simulink model "trucksim_different_condition"  (R2023b)
settings: Solver=FixedStepAuto  StartTime=0.0  StopTime=25  FixedStep=0.001  RelTol=1e-3  EnableMultiTasking=on
values from neighbouring files (symbols this model uses):
  g = 9.8    [Truck_simulate_different_condition.m]
  m = m_sprung + m_load + m_unsprung    (= 10505)    [Truck_simulate_different_condition.m]
  r = 0.510    (= 0.51)    [Truck_simulate_different_condition.m]
  vx0 = 5    [Truck_simulate_different_condition.m]
  vy0 = 0    [Truck_simulate_different_condition.m]
  w0 = vx0 / r    (= 9.80392156863)    [Truck_simulate_different_condition.m]
  wz0 = 0    [Truck_simulate_different_condition.m]
undefined symbols (not defined in the file or in its folder): A, Bf, Br, Cd, Cs_f, f, He, hg, Hp, I_tire, Ix, Iy, Iz, ks_f, kw, L, Lf, Lr, mb, mw, p
libraries: SignalEditorBlockLib x6, Solver_SF x1
(part 1 of 4)
settings Model: Creator=dzY  LastModifiedBy=Admin
settings DataIOCC: SaveFormat=Array  ReturnWorkspaceOutputs=off
settings OptimizationCC: LifeSpan=inf
settings DebuggingCC: SolverPrmCheckMsg=warning  UnconnectedInputMsg=warning  UnconnectedOutputMsg=warning  UnconnectedLineMsg=warning  SFUnexpectedBacktrackingDiag=warning  SFNoUnconditionalDefaultTransitionDiag=warning  SFExecutionAtInitializationDiag=none  ArithmeticOperatorsInVariantConditions=warning
settings HardwareCC: ProdBitPerPointer=32  ProdBitPerSizeT=32  ProdBitPerPtrDiffT=32  ProdLargestAtomicFloat=None  ProdIntDivRoundTo=Undefined  ProdEndianess=Unspecified  ProdWordSize=32  ProdHWDeviceType=32-bit Generic
settings ModelReferenceCC: EnableRefExpFcnMdlSchedulingChecks=on  PropagateSignalLabelsOutOfModel=off
settings SFSimCC: SimUseLocalCustomCode=off  CustomCodeUndefinedFunction=UseInterfaceOnly
settings RTWCC: RTWUseLocalCustomCode=off
settings CodeAppCC: StateflowObjectComments=on
settings GRTTargetCC: TargetLangStandard=C89/C90 (ANSI)
settings ConfigComp: CovMetricSettings=dw  CovSaveCumulativeToWorkspaceVar=on  CovSaveSingleToWorkspaceVar=on  CovExternalEMLEnable=off  CovSFcnEnable=off

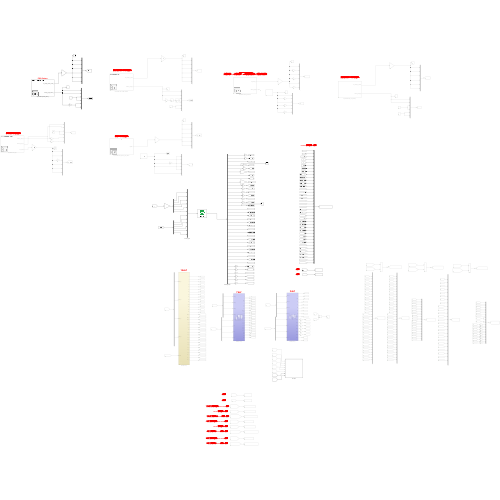
[thumbnail: Simulink's stored preview of the top-level diagram]
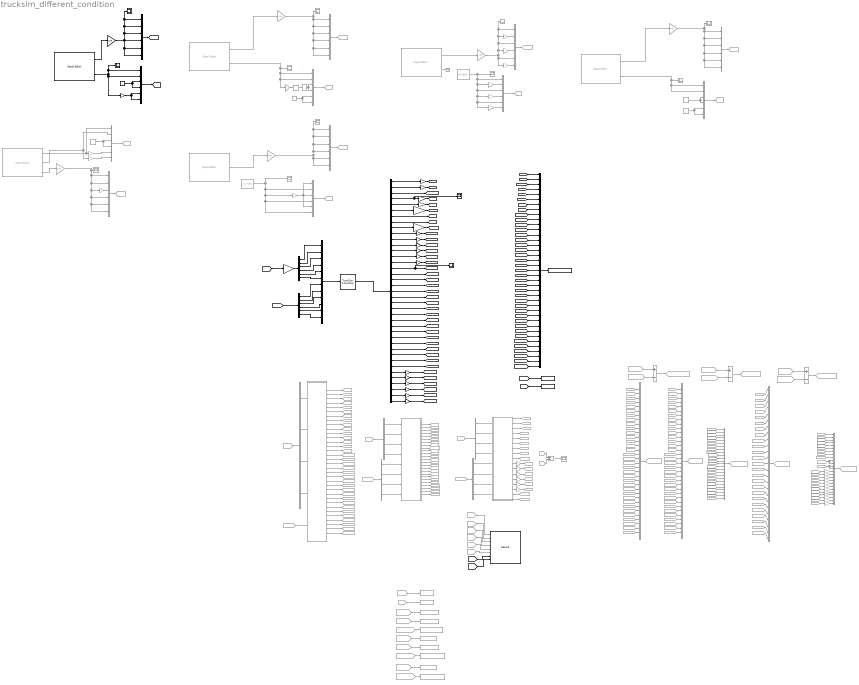
== system trucksim_different_condition ==
  note: FRO Pattern
  note: 原地掉头控制输入
  note: 7dof
  note: 4维度
  note: 4维度
  note: 十四自由度模型输出18+4+12=34维度
  note: carsim模型输出34维度
  note: 十四自由度模型与carsim残差34维度
  note: carsim模型输出25维度
  note: 七自由度模型与carsim残差25维度
  note: 七自由度模型输出18+4+12=25维度
  note: 14dof
  note: 3dof
  note: 三自由度模型与carsim残差25维度
  note: 三自由度模型输出18+4+12=25维度
  note: 6维度
  note: trucksim模型输出39维度
  note: 6维度
  note: 前中轴转向工况控制输入
  note: 蟹形工况控制输入
  note: 横移工况控制输入
      | (左侧左转90，右侧右转90，左侧前进转矩，右侧后退转矩)
  note: 仅前轴转向工况控制输入
  14DOF整车模型 : Subsystem  Commented=on
  3DOF整车模型 : Subsystem  Commented=on
  7DOF整车模型 : Subsystem  Commented=on
  Add{,1..3} (4 alike) : Sum  Commented=on  Inputs=+-
  Constant{,3,5..6} (4 alike) : Constant  Commented=on  Value=0
  Constant1 : Constant  Value=0
  Constant2 : Constant  Commented=on  Value=3.1415/2
  Constant4 : Constant  Commented=on  Value=3.14159/2
  Demux{,2,4..6} (5 alike) : Demux  Commented=on
  Demux1 : Demux  Outputs=6
  Demux3 : Demux  Outputs=6
  From{,32,82,89} (4 alike) : From  Commented=on  GotoTag=delta_act
  From1 : From  Commented=on  GotoTag=x_14dof
  From10 : From  Commented=on  GotoTag=ay_14dof
  From100 : From  Commented=on  GotoTag=Fy_fl_7dof
  From101 : From  Commented=on  GotoTag=Fz_fl_7dof
  From102 : From  Commented=on  GotoTag=Fx_fr_7dof
  From103 : From  Commented=on  GotoTag=Fy_fr_7dof
  From104 : From  Commented=on  GotoTag=Fz_fr_7dof
  From105 : From  Commented=on  GotoTag=Fx_rl_7dof
  From106 : From  Commented=on  GotoTag=Fy_rl_7dof
  From107 : From  Commented=on  GotoTag=Fz_rl_7dof
  From108 : From  Commented=on  GotoTag=Fx_rr_7dof
  From109 : From  Commented=on  GotoTag=Fy_rr_7dof
  From11 : From  Commented=on  GotoTag=az_14dof
  From110 : From  Commented=on  GotoTag=Fz_rr_7dof
  From111 : From  Commented=on  GotoTag=Fx_fl_carsim
  From112 : From  Commented=on  GotoTag=Fy_fl_carsim
  From113 : From  Commented=on  GotoTag=x_carsim
  From114 : From  Commented=on  GotoTag=y_carsim
  From115 : From  Commented=on  GotoTag=state_7dof_25d
  From116 : From  Commented=on  GotoTag=vx_carsim
  From117 : From  Commented=on  GotoTag=state_carsim_25d
  From118 : From  Commented=on  GotoTag=vy_carsim
  From119 : From  Commented=on  GotoTag=ax_carsim
  From12 : From  Commented=on  GotoTag=roll_14dof
  From120 : From  Commented=on  GotoTag=ay_carsim
  From121 : From  Commented=on  GotoTag=state_7dof_25d
  From122 : From  Commented=on  GotoTag=state_residual_7dof_25d
  From123 : From  Commented=on  GotoTag=state_carsim_25d
  From124 : From  Commented=on  GotoTag=yaw_carsim
  From125 : From  Commented=on  GotoTag=Fy_f_3dof
  From126 : From  Commented=on  GotoTag=Fz_f_3dof
  From127 : From  Commented=on  GotoTag=wz_carsim
  From128 : From  Commented=on  GotoTag=Fy_r_3dof
  From129 : From  Commented=on  GotoTag=Fz_r_3dof
  From13 : From  Commented=on  GotoTag=phi_14dof
  From130 : From  Commented=on  GotoTag=beta_z_carsim
  From131 : From  Commented=on  GotoTag=w_fl_carsim
  From132 : From  Commented=on  GotoTag=w_fr_carsim
  From133 : From  Commented=on  GotoTag=w_rl_carsim
  From134 : From  Commented=on  GotoTag=w_rr_carsim
  From135 : From  Commented=on  GotoTag=Fz_fl_carsim
  From136 : From  Commented=on  GotoTag=Fx_fr_carsim
  From137 : From  Commented=on  GotoTag=Fy_fr_carsim
  From138 : From  Commented=on  GotoTag=Fz_fr_carsim
  From139 : From  Commented=on  GotoTag=Fx_rl_carsim
  From140 : From  Commented=on  GotoTag=Fy_rl_carsim
  From141 : From  Commented=on  GotoTag=Fz_rl_carsim
  From142 : From  Commented=on  GotoTag=Fx_rr_carsim
  From143 : From  Commented=on  GotoTag=Fy_rr_carsim
  From144 : From  Commented=on  GotoTag=Fz_rr_carsim
  From145 : From  Commented=on  GotoTag=Fx_r_3dof
  From146 : From  Commented=on  GotoTag=Fy_r_3dof
  From147 : From  Commented=on  GotoTag=Fz_r_3dof
  From148 : From  Commented=on  GotoTag=Fx_r_3dof
  From149 : From  Commented=on  GotoTag=w_f_3dof
  From15 : From  Commented=on  GotoTag=yaw_14dof
  From150 : From  Commented=on  GotoTag=state_3dof_25d
  From151 : From  Commented=on  GotoTag=w_r_3dof
  From152 : From  Commented=on  GotoTag=state_3dof_25d
  From153 : From  Commented=on  GotoTag=x_3dof
  From154 : From  Commented=on  GotoTag=y_3dof
  From155 : From  Commented=on  GotoTag=yaw_3dof
  From156 : From  Commented=on  GotoTag=vx_3dof
  From157 : From  Commented=on  GotoTag=vy_3dof
  From158 : From  Commented=on  GotoTag=wz_3dof
  From159 : From  Commented=on  GotoTag=ax_3dof
  From16 : From  Commented=on  GotoTag=wx_14dof
  From160 : From  Commented=on  GotoTag=ay_3dof
  From161 : From  Commented=on  GotoTag=beta_z_3dof
  From162 : From  Commented=on  GotoTag=Fx_f_3dof
  From163 : From  Commented=on  GotoTag=state_carsim_25d
  From164 : From  Commented=on  GotoTag=state_residual_3dof_25d
  From165 : From  Commented=on  GotoTag=x_14dof
  From166 : From  Commented=on  GotoTag=y_14dof
  From167 : From  Commented=on  GotoTag=x_7dof
  From168 : From  Commented=on  GotoTag=y_7dof
  From169 : From  Commented=on  GotoTag=x_3dof
  From17 : From  Commented=on  GotoTag=wy_14dof
  From170 : From  Commented=on  GotoTag=y_3dof
  From173 : From  Commented=on  GotoTag=vx_14dof
  From174 : From  Commented=on  GotoTag=vx_carsim
  From18 : From  Commented=on  GotoTag=wz_14dof
  From19 : From  Commented=on  GotoTag=beta_x_14dof
  From2 : From  Commented=on  GotoTag=y_14dof
  From20 : From  Commented=on  GotoTag=beta_y_14dof
  From21 : From  Commented=on  GotoTag=beta_z_14dof
  From22 : From  Commented=on  GotoTag=w_fl_14dof
  From23 : From  Commented=on  GotoTag=w_fr_14dof
  From24 : From  Commented=on  GotoTag=w_rl_14dof
  From25 : From  Commented=on  GotoTag=w_rr_14dof
  From26 : From  Commented=on  GotoTag=state_carsim_34d
  From27 : From  Commented=on  GotoTag=state_14dof_34d
  From28 : From  Commented=on  GotoTag=w_fl_7dof
  From29 : From  Commented=on  GotoTag=w_fr_7dof
  From30 : From  Commented=on  GotoTag=w_rl_7dof
  From{4,31,81,88} (4 alike) : From  Commented=on  GotoTag=T_motor
  From33 : From  Commented=on  GotoTag=Fy_f_3dof
  From34 : From  Commented=on  GotoTag=Fz_f_3dof
  From35 : From  Commented=on  GotoTag=Fx_fl_carsim
  From36 : From  Commented=on  GotoTag=Fy_fl_carsim
  From37 : From  Commented=on  GotoTag=x_carsim
  From38 : From  Commented=on  GotoTag=y_carsim
  From39 : From  Commented=on  GotoTag=z_carsim
  From40 : From  Commented=on  GotoTag=vx_carsim
  From41 : From  Commented=on  GotoTag=vz_carsim
  From42 : From  Commented=on  GotoTag=vy_carsim
  From43 : From  Commented=on  GotoTag=ax_carsim
  From44 : From  Commented=on  GotoTag=ay_carsim
  From45 : From  Commented=on  GotoTag=az_carsim
  From46 : From  Commented=on  GotoTag=roll_carsim
  From47 : From  Commented=on  GotoTag=phi_carsim
  From48 : From  Commented=on  GotoTag=yaw_carsim
  From49 : From  Commented=on  GotoTag=wx_carsim
  From5 : From  Commented=on  GotoTag=z_14dof
  From50 : From  Commented=on  GotoTag=wy_carsim
  From51 : From  Commented=on  GotoTag=wz_carsim
  From52 : From  Commented=on  GotoTag=beta_x_carsim
  From53 : From  Commented=on  GotoTag=beta_y_carsim
  From54 : From  Commented=on  GotoTag=beta_z_carsim
  From55 : From  Commented=on  GotoTag=w_fl_carsim
  From56 : From  Commented=on  GotoTag=w_fr_carsim
  From57 : From  Commented=on  GotoTag=w_rl_carsim
  From58 : From  Commented=on  GotoTag=w_rr_carsim
  From59 : From  Commented=on  GotoTag=Fz_fl_carsim
  From6 : From  Commented=on  GotoTag=vx_14dof
  From60 : From  Commented=on  GotoTag=Fx_fr_carsim
  From61 : From  Commented=on  GotoTag=Fy_fr_carsim
  From62 : From  Commented=on  GotoTag=Fz_fr_carsim
  From63 : From  Commented=on  GotoTag=Fx_rl_carsim
  From64 : From  Commented=on  GotoTag=Fy_rl_carsim
  From65 : From  Commented=on  GotoTag=Fz_rl_carsim
  From66 : From  Commented=on  GotoTag=Fx_rr_carsim
  From67 : From  Commented=on  GotoTag=Fy_rr_carsim
  From68 : From  Commented=on  GotoTag=Fz_rr_carsim
  From69 : From  Commented=on  GotoTag=Fx_fl_14dof
  From7 : From  Commented=on  GotoTag=vy_14dof
  From70 : From  Commented=on  GotoTag=Fy_fl_14dof
  From71 : From  Commented=on  GotoTag=Fz_fl_14dof
  From72 : From  Commented=on  GotoTag=Fx_fr_14dof
  From73 : From  Commented=on  GotoTag=Fy_fr_14dof
  From74 : From  Commented=on  GotoTag=Fz_fr_14dof
  From75 : From  Commented=on  GotoTag=Fx_rl_14dof
  From76 : From  Commented=on  GotoTag=Fy_rl_14dof
  From77 : From  Commented=on  GotoTag=Fz_rl_14dof
  From78 : From  Commented=on  GotoTag=Fx_rr_14dof
  From79 : From  Commented=on  GotoTag=Fy_rr_14dof
  From8 : From  Commented=on  GotoTag=vz_14dof
  From80 : From  Commented=on  GotoTag=Fz_rr_14dof
  From83 : From  Commented=on  GotoTag=state_14dof_34d
  From84 : From  Commented=on  GotoTag=state_residual_14dof_34d
  From85 : From  Commented=on  GotoTag=w_rr_7dof
  From86 : From  Commented=on  GotoTag=Fx_f_3dof
  From87 : From  Commented=on  GotoTag=state_carsim_34d
  From9 : From  Commented=on  GotoTag=ax_14dof
  From90 : From  Commented=on  GotoTag=x_7dof
  From91 : From  Commented=on  GotoTag=y_7dof
  From92 : From  Commented=on  GotoTag=yaw_7dof
  From93 : From  Commented=on  GotoTag=vx_7dof
  From94 : From  Commented=on  GotoTag=vy_7dof
  From95 : From  Commented=on  GotoTag=wz_7dof
  From96 : From  Commented=on  GotoTag=ax_7dof
  From97 : From  Commented=on  GotoTag=ay_7dof
  From98 : From  Commented=on  GotoTag=beta_z_7dof
  From99 : From  Commented=on  GotoTag=Fx_fl_7dof
  Gain : Gain  Gain=1/3.6
  Gain{1,39,43,46,48..53} (10 alike) : Gain  Commented=on  Gain=-1
  Gain{8..10,12,35..38} (8 alike) : Gain  Gain=3.1415/180
  Gain{11,18..22} (6 alike) : Gain  Commented=on  Gain=2
  Gain{3,6,13..16} (6 alike) : Gain  Gain=3.1415/30
  Gain17 : Gain  Gain=180/3.1415
  Gain2 : Gain  Gain=1/3.6
  Gain{23..34,45} (13 alike) : Gain  Commented=on  Gain=0.5
  Gain4 : Gain  Gain=9.8
  Gain40 : Gain  Gain=-1
  Gain{7,41,44,47,54} (5 alike) : Gain  Commented=on  Gain=100
  Gain42 : Gain  Gain=100
  Gain5 : Gain  Gain=9.8
  Goto{,127,129,131,133} (5 alike) : Goto  Commented=on  GotoTag=delta_act
  Goto1 : Goto  Commented=on  GotoTag=w_fl_14dof
  Goto100 : Goto  Commented=on  GotoTag=state_residual_7dof_25d
  Goto101 : Goto  Commented=on  GotoTag=wz_3dof
  Goto102 : Goto  Commented=on  GotoTag=ax_3dof
  Goto103 : Goto  Commented=on  GotoTag=vy_3dof
  Goto104 : Goto  Commented=on  GotoTag=vx_3dof
  Goto105 : Goto  Commented=on  GotoTag=Fx_f_3dof
  Goto106 : Goto  Commented=on  GotoTag=Fy_f_3dof
  Goto107 : Goto  Commented=on  GotoTag=Fz_f_3dof
  Goto108 : Goto  Commented=on  GotoTag=state_3dof_25d
  Goto109 : Goto  Commented=on  GotoTag=state_residual_3dof_25d
  Goto111 : Goto  Commented=on  GotoTag=Fx_r_3dof
  Goto112 : Goto  Commented=on  GotoTag=Fy_r_3dof
  Goto113 : Goto  Commented=on  GotoTag=Fz_r_3dof
  Goto117 : Goto  Commented=on  GotoTag=ay_3dof
  Goto118 : Goto  Commented=on  GotoTag=beta_z_3dof
  Goto119 : Goto  Commented=on  GotoTag=x_3dof
  Goto120 : Goto  Commented=on  GotoTag=y_3dof
  Goto121 : Goto  Commented=on  GotoTag=yaw_3dof
  Goto122 : Goto  Commented=on  GotoTag=w_f_3dof
  Goto124 : Goto  Commented=on  GotoTag=w_r_3dof
  Goto{38,128,130,132,134} (5 alike) : Goto  Commented=on  GotoTag=T_motor
  Goto2 : Goto  Commented=on  GotoTag=x_14dof
  Goto3 : Goto  Commented=on  GotoTag=y_14dof
  Goto31 : Goto  Commented=on  GotoTag=state_carsim_34d
  Goto32 : Goto  Commented=on  GotoTag=state_14dof_34d
  Goto33 : Goto  Commented=on  GotoTag=state_residual_14dof_34d
  Goto34 : Goto  Commented=on  GotoTag=wz_7dof
  Goto4 : Goto  Commented=on  GotoTag=z_14dof
  Goto48 : Goto  Commented=on  GotoTag=Fx_fl_14dof
  Goto49 : Goto  Commented=on  GotoTag=vy_14dof
  Goto5 : Goto  Commented=on  GotoTag=vx_14dof
  Goto50 : Goto  Commented=on  GotoTag=vz_14dof
  Goto51 : Goto  Commented=on  GotoTag=ax_14dof
  Goto52 : Goto  Commented=on  GotoTag=ay_14dof
  Goto53 : Goto  Commented=on  GotoTag=az_14dof
  Goto54 : Goto  Commented=on  GotoTag=roll_14dof
  Goto55 : Goto  Commented=on  GotoTag=phi_14dof
  Goto56 : Goto  Commented=on  GotoTag=yaw_14dof
  Goto57 : Goto  Commented=on  GotoTag=wx_14dof
  Goto58 : Goto  Commented=on  GotoTag=wy_14dof
  Goto59 : Goto  Commented=on  GotoTag=wz_14dof
  Goto6 : Goto  Commented=on  GotoTag=w_fr_14dof
  Goto60 : Goto  Commented=on  GotoTag=beta_x_14dof
  Goto61 : Goto  Commented=on  GotoTag=beta_y_14dof
  Goto62 : Goto  Commented=on  GotoTag=beta_z_14dof
  Goto63 : Goto  Commented=on  GotoTag=Fy_fl_14dof
  Goto64 : Goto  Commented=on  GotoTag=Fz_fl_14dof
  Goto65 : Goto  Commented=on  GotoTag=Fx_fr_14dof
  Goto66 : Goto  Commented=on  GotoTag=Fy_fr_14dof
  Goto67 : Goto  Commented=on  GotoTag=Fz_fr_14dof
  Goto68 : Goto  Commented=on  GotoTag=Fx_rl_14dof
  Goto69 : Goto  Commented=on  GotoTag=Fy_rl_14dof
  Goto7 : Goto  Commented=on  GotoTag=w_rl_14dof
  Goto70 : Goto  Commented=on  GotoTag=Fz_rl_14dof
  Goto71 : Goto  Commented=on  GotoTag=Fx_rr_14dof
  Goto72 : Goto  Commented=on  GotoTag=Fy_rr_14dof
  Goto73 : Goto  Commented=on  GotoTag=Fz_rr_14dof
  Goto74 : Goto  Commented=on  GotoTag=ax_7dof
  Goto75 : Goto  Commented=on  GotoTag=vy_7dof
  Goto76 : Goto  Commented=on  GotoTag=vx_7dof
  Goto77 : Goto  Commented=on  GotoTag=Fx_fl_7dof
  Goto78 : Goto  Commented=on  GotoTag=Fy_fl_7dof
  Goto79 : Goto  Commented=on  GotoTag=Fz_fl_7dof
  Goto8 : Goto  Commented=on  GotoTag=w_rr_14dof
  Goto80 : Goto  Commented=on  GotoTag=Fx_fr_7dof
  Goto81 : Goto  Commented=on  GotoTag=Fy_fr_7dof
  Goto82 : Goto  Commented=on  GotoTag=Fz_fr_7dof
  Goto83 : Goto  Commented=on  GotoTag=Fx_rl_7dof
  Goto84 : Goto  Commented=on  GotoTag=Fy_rl_7dof
  Goto85 : Goto  Commented=on  GotoTag=Fz_rl_7dof
  Goto86 : Goto  Commented=on  GotoTag=Fx_rr_7dof
  Goto87 : Goto  Commented=on  GotoTag=Fy_rr_7dof
  Goto88 : Goto  Commented=on  GotoTag=Fz_rr_7dof
  Goto89 : Goto  Commented=on  GotoTag=ay_7dof
  Goto90 : Goto  Commented=on  GotoTag=beta_z_7dof
  Goto91 : Goto  Commented=on  GotoTag=x_7dof
  Goto92 : Goto  Commented=on  GotoTag=y_7dof
  Goto93 : Goto  Commented=on  GotoTag=yaw_7dof
  Goto94 : Goto  Commented=on  GotoTag=state_7dof_25d
  Goto95 : Goto  Commented=on  GotoTag=w_fl_7dof
  Goto96 : Goto  Commented=on  GotoTag=w_fr_7dof
  Goto97 : Goto  Commented=on  GotoTag=w_rl_7dof
  Goto98 : Goto  Commented=on  GotoTag=w_rr_7dof
  Goto99 : Goto  Commented=on  GotoTag=state_carsim_25d
  Mux{,4,10..17} (10 alike) : Mux  Commented=on  Inputs=6
  Mux1 : Mux  Commented=on  Inputs=34
  Mux2 : Mux  Commented=on  Inputs=34
  Mux3 : Mux  Commented=on  Inputs=25
  Mux5 : Mux  Commented=on  Inputs=25
  Mux6 : Mux  Commented=on  Inputs=25
  Mux7 : Mux  Inputs=39
  Mux8 : Mux  Inputs=6
  Mux9 : Mux  Inputs=6
  Scope{,4..5,7..13} (10 alike) : Scope  Commented=on
  Scope{1..3,6} (4 alike) : Scope
  Signal Editor-front_middle_steering : SignalEditorBlockLib/Signal Editor  Commented=on  FileName=D:\YRJ_Workspace\Dynamic_Model_with_NN_truck\data\trucksim\different_scenarios\scenarios_input\Scenario-input_front_middle_steering_v1.mat  ActiveScenario=Scenario_snake_deacc_5m_s_16  ActiveSignal=tire_torque_4_deacc  IsBus=off  OutputBusObjectStr=Bus: BusObject  SampleTime=0  ZeroCross=off  OutputAfterFinalValue=Setting to zero  Unit=inherit  PreserveSignalName=on  ApplySigPropsToAllScenarios=on  ApplySigPropsToAllSignals=on
  Signal Editor-lateral_movement : SignalEditorBlockLib/Signal Editor  Commented=on  FileName=D:\YRJ_Workspace\Dynamic_Model_with_NN_truck\data\trucksim\different_scenarios\scenarios_input\Scenario-input_lateral_movement_v1.mat  ActiveScenario=Scenario_lateral_movement_6  ActiveSignal=tire_torque_6  IsBus=off  OutputBusObjectStr=Bus: BusObject  SampleTime=0  ZeroCross=off  OutputAfterFinalValue=Setting to zero  Unit=inherit  PreserveSignalName=on  ApplySigPropsToAllScenarios=on  ApplySigPropsToAllSignals=on
  Signal Editor-only_front_steering : SignalEditorBlockLib/Signal Editor  Commented=on  FileName=D:\YRJ_Workspace\Dynamic_Model_with_NN_truck\data\trucksim\different_scenarios\scenarios_input\Scenario-input_front_middle_steering_v1.mat  ActiveScenario=Scenario_snake_deacc_5m_s_16  ActiveSignal=tire_torque_4_deacc  IsBus=off  OutputBusObjectStr=Bus: BusObject  SampleTime=0  ZeroCross=off  OutputAfterFinalValue=Setting to zero  Unit=inherit  PreserveSignalName=on  ApplySigPropsToAllScenarios=on  ApplySigPropsToAllSignals=on
  Signal Editor-opposite_steering : SignalEditorBlockLib/Signal Editor  FileName=D:\YRJ_Workspace\Dynamic_Model_with_NN_truck\data\trucksim\different_scenarios\scenarios_input\Scenario-input_snake_rollover_v2_5m_s.mat  ActiveScenario=Scenario_snake_rollover_5m_s_1  ActiveSignal=tire_torque_rollover_const_1  IsBus=off  OutputBusObjectStr=Bus: BusObject  SampleTime=0  ZeroCross=off  OutputAfterFinalValue=Setting to zero  Unit=inherit  PreserveSignalName=on  ApplySigPropsToAllScenarios=on  ApplySigPropsToAllSignals=on
  Signal Editor-same_steering_crab_motion : SignalEditorBlockLib/Signal Editor  Commented=on  FileName=D:\YRJ_Workspace\Dynamic_Model_with_NN_truck\data\trucksim\different_scenarios\scenarios_input\Scenario-input_same_steering_lateral_movement_v1.mat  ActiveScenario=Scenario_lateral_movement_6  ActiveSignal=tire_torque_6  IsBus=off  OutputBusObjectStr=Bus: BusObject  SampleTime=0  ZeroCross=off  OutputAfterFinalValue=Setting to zero  Unit=inherit  PreserveSignalName=on  ApplySigPropsToAllScenarios=on  ApplySigPropsToAllSignals=on
  Signal Editor-tank_turn : SignalEditorBlockLib/Signal Editor  Commented=on  FileName=D:\YRJ_Workspace\Dynamic_Model_with_NN_truck\data\trucksim\different_scenarios\scenarios_input\Scenario-input_tank_turn_v1.mat  ActiveScenario=Scenario_tank_turn_1500Nm  ActiveSignal=steering_angle_fl  IsBus=off  OutputBusObjectStr=Bus: BusObject  SampleTime=0  ZeroCross=off  OutputAfterFinalValue=Setting to zero  Unit=inherit  PreserveSignalName=on  ApplySigPropsToAllScenarios=on  ApplySigPropsToAllSignals=on
  Terminator1 : Terminator  Commented=on
  To Workspace1 : ToWorkspace  Commented=on  VariableName=T_motor_out  SaveFormat=Timeseries  SampleTime=-1
  To Workspace10 : ToWorkspace  Commented=on  VariableName=Vehicle_state_residual_3dof_25d_out  SaveFormat=Timeseries  SampleTime=-1
  To Workspace11 : ToWorkspace  VariableName=Vehicle_state_trucksim_39d_out  SaveFormat=Timeseries  SampleTime=-1
  To Workspace12 : ToWorkspace  VariableName=T_motor_out  SaveFormat=Timeseries  SampleTime=-1
  To Workspace13 : ToWorkspace  VariableName=Delta_act_out  SaveFormat=Timeseries  SampleTime=-1
  To Workspace2 : ToWorkspace  Commented=on  VariableName=Vehicle_state_7dof_25d_out  SaveFormat=Timeseries  SampleTime=-1
  To Workspace3 : ToWorkspace  Commented=on  VariableName=Delta_act_out  SaveFormat=Timeseries  SampleTime=-1
  To Workspace4 : ToWorkspace  Commented=on  VariableName=Vehicle_state_14dof_34d_out  SaveFormat=Timeseries  SampleTime=-1
  To Workspace5 : ToWorkspace  Commented=on  VariableName=Vehicle_state_residual_14dof_34d_out  SaveFormat=Timeseries  SampleTime=-1
  To Workspace6 : ToWorkspace  Commented=on  VariableName=Vehicle_state_carsim_34d_out  SaveFormat=Timeseries  SampleTime=-1
  To Workspace7 : ToWorkspace  Commented=on  VariableName=Vehicle_state_residual_7dof_25d_out  SaveFormat=Timeseries  SampleTime=-1
  To Workspace8 : ToWorkspace  Commented=on  VariableName=Vehicle_state_carsim_25d_out  SaveFormat=Timeseries  SampleTime=-1
  To Workspace9 : ToWorkspace  Commented=on  VariableName=Vehicle_state_3dof_25d_out  SaveFormat=Timeseries  SampleTime=-1
  Trigonometric Function : Trigonometry  Commented=on  Operator=tan
  Trigonometric Function1 : Trigonometry  Commented=on  Operator=atan
  TruckSim S-Function : Solver_SF/TruckSim S-Function  Priority=1  SIMFILE=simfile.sim
      settings: SourceProductName=TruckSim S-Function
  Trucksim_Input : Mux  Inputs=12
  Trucksim_Output : Demux  Outputs=39
  XY Graph : Record  FileSettingsInternal="{\"entries\":[{\"content\":{\"excelSettings\":{\"content\":{},\"type\":\"Streamout.ExcelSettings\"}},\"type\":\"Streamout.FileSettingStorage\",\"uuid\":\"\"}],\"packageUris\":[\"http:\\/\\/schema.mathworks.com\\/mf0\\/streamout_blocks\\/R2020a\"],\"version\":\"1.0\"}"  Layout=[1 1]  SignalsInternal="{\"entries\":[{\"content\":{\"signals\":[{\"content\":{\"blockPath\":[],\"dimensions\":[1],\"domain\":\"\",\"lineColor\":\"#d95319\",\"port\":1,\"signalID\":8,\"signalName\":\"From165\"},\"type\":\"RecordBlkView.Signal\",\"uuid\":\"\"},{\"content\":{\"blockPath\":[],\"dimensions\":[1],\"domain\":\"\",\"lineColor\":\"#edb120\",\"port\":2,\"signalID\":11,\"signalName\":\"From166\"},\"type\":\"RecordBlkView.Signal\",\"uuid\":\"\"},{\"content\":{\"blockPath\":[],\"dimensions\":[1],\"domain\":\"\",\"lineColor\":\"#7e2f8e\",\"port\":3,\"signalID\":14,\"signalName\":\"From167\"},\"type\":\"RecordBlkView.Signal\",\"uuid\":\"\"},{\"content\":{\"blockPath\":[],\"dimensions\":[1],\"domain\":\"\",\"lineColor\":\"#77ac30\",\"port\":4,\"signalID\":17,\"signalName\":\"From168\"},\"type\":\"RecordBlkView.Signal\",\"uuid\":\"\"},{\"content\":{\"blockPath\":[],\"dimensions\":[1],\"domain\":\"\",\"lineColor\":\"#4dbeee\",\"port\":5,\"signalID\":20,\"signalName\":\"From169\"},\"type\":\"RecordBlkView.Signal\",\"uuid\":\"\"},{\"content\":{\"blockPath\":[],\"dimensions\":[1],\"domain\":\"\",\"lineColor\":\"#a2142f\",\"port\":6,\"signalID\":23,\"signalName\":\"From170\"},\"type\":\"RecordBlkView.Signal\",\"uuid\":\"\"},{\"content\":{\"blockPath\":[],\"dimensions\":[1],\"domain\":\"\",\"lineColor\":\"#139fff\",\"port\":7,\"signalID\":26,\"signalName\":\"From171\"},\"type\":\"RecordBlkView.Signal\",\"uuid\":\"\"},{\"content\":{\"blockPath\":[],\"dimensions\":[1],\"domain\":\"\",\"lineColor\":\"#ff6929\",\"port\":8,\"signalID\":29,\"signalName\":\"From172\"},\"type\":\"RecordBlkView.Signal\",\"uuid\":\"\"}]},\"type\":\"RecordBlkView.InputSignals\",\"uuid\":\"\"}],\"packageUris\":[\"http:\\/\\/schema.mathworks.com\\/mf0\\/streamout_blocks\\/R2020a\"],\"version\":\"1.0\"}"  VisualizationBindings="{\"xyplotplugin\":{\"info\":[{\"series\":[],\"subplotID\":1}]}}"  CompatibilityTag=XY
  wires:
  From4/1 -> 14DOF整车模型/5(Pedal)
  Mux4/1 -> Goto38/1
  14DOF整车模型/1(x) -> Goto2/1
  14DOF整车模型/2(y) -> Goto3/1
  14DOF整车模型/3(z) -> Goto4/1
  14DOF整车模型/4(vx) -> Goto5/1
  14DOF整车模型/5(vy) -> Goto49/1
  14DOF整车模型/6(vz) -> Goto50/1
  14DOF整车模型/7(ax) -> Goto51/1
  14DOF整车模型/8(ay) -> Goto52/1
  14DOF整车模型/9(az) -> Goto53/1
  14DOF整车模型/10(roll) -> Goto54/1
  14DOF整车模型/11(phi) -> Goto55/1
  14DOF整车模型/12(yaw) -> Goto56/1
  14DOF整车模型/13(wx) -> Goto57/1
  14DOF整车模型/14(wy) -> Goto58/1
  14DOF整车模型/15(wz) -> Goto59/1
  14DOF整车模型/16(beta_x) -> Goto60/1
  14DOF整车模型/17(beta_y) -> Goto61/1
  14DOF整车模型/18(beta_z) -> Goto62/1
  From1/1 -> Mux2/1
  From2/1 -> Mux2/2
  From5/1 -> Mux2/3
  From6/1 -> Mux2/4
  From7/1 -> Mux2/5
  From8/1 -> Mux2/6
  From9/1 -> Mux2/7
  From10/1 -> Mux2/8
  From11/1 -> Mux2/9
  From12/1 -> Mux2/10
  From13/1 -> Mux2/11
  From15/1 -> Mux2/12
  From16/1 -> Mux2/13
  From17/1 -> Mux2/14
  From18/1 -> Mux2/15
  From19/1 -> Mux2/16
  From20/1 -> Mux2/17
  From21/1 -> Mux2/18
  Mux2/1 -> Goto32/1
  Mux/1 -> Goto/1
  Gain1/1 -> Mux/5
  Demux/4 -> 14DOF整车模型/4(delta_rr)
  Demux/3 -> 14DOF整车模型/3(delta_rl)
  Demux/2 -> 14DOF整车模型/2(delta_fr)
  Demux/1 -> 14DOF整车模型/1(delta_fl)
  From/1 -> Demux/1
  Demux1/2 -> Trucksim_Input/2
  Demux1/1 -> Trucksim_Input/1
  14DOF整车模型/19(w_fl) -> Goto1/1
  14DOF整车模型/20(w_fr) -> Goto6/1
  14DOF整车模型/21(w_rl) -> Goto7/1
  14DOF整车模型/22(wrr) -> Goto8/1
  From22/1 -> Mux2/19
  From23/1 -> Mux2/20
  From24/1 -> Mux2/21
  From25/1 -> Mux2/22
  From27/1 -> Add/2
  From26/1 -> Add/1
  Add/1 -> Goto33/1
  Gain2/1 -> [vy_trucksim]
  Gain/1 -> [vx_trucksim]
  Gain9/1 -> [yaw_trucksim]
  Gain12/1 -> [wz_trucksim]
  Gain13/1 -> [w_fl_trucksim]
  Gain14/1 -> [w_fr_trucksim]
  Gain15/1 -> [w_rl_trucksim]
  Gain16/1 -> [w_rr_trucksim]
  Gain17/1 -> Demux1/1
  [delta_act] -> Gain17/1
  From37/1 -> Mux1/1
  From38/1 -> Mux1/2
  From39/1 -> Mux1/3
  From40/1 -> Mux1/4
  From42/1 -> Mux1/5
  From41/1 -> Mux1/6
  From43/1 -> Mux1/7
  From44/1 -> Mux1/8
  From45/1 -> Mux1/9
  From46/1 -> Mux1/10
  From47/1 -> Mux1/11
  From48/1 -> Mux1/12
  From49/1 -> Mux1/13
  From50/1 -> Mux1/14
  From51/1 -> Mux1/15
  From52/1 -> Mux1/16
  From53/1 -> Mux1/17
  From54/1 -> Mux1/18
  From55/1 -> Mux1/19
  From56/1 -> Mux1/20
  From57/1 -> Mux1/21
  From58/1 -> Mux1/22
  Mux1/1 -> Goto31/1
  From35/1 -> Mux1/23
  From36/1 -> Mux1/24
  From59/1 -> Mux1/25
  From60/1 -> Mux1/26
  From61/1 -> Mux1/27
  From62/1 -> Mux1/28
  From63/1 -> Mux1/29
  From64/1 -> Mux1/30
  From65/1 -> Mux1/31
  From66/1 -> Mux1/32
  From67/1 -> Mux1/33
  From68/1 -> Mux1/34
  14DOF整车模型/23(Fx_fl) -> Goto48/1
  14DOF整车模型/24(Fy_fl) -> Goto63/1
  14DOF整车模型/25(Fz_fl) -> Goto64/1
  14DOF整车模型/26(Fx_fr) -> Goto65/1
  14DOF整车模型/27(Fy_fr) -> Goto66/1
  14DOF整车模型/28(Fz_fr) -> Goto67/1
  14DOF整车模型/29(Fx_rl) -> Goto68/1
  14DOF整车模型/30(Fy_rl) -> Goto69/1
  14DOF整车模型/31(Fz_rl) -> Goto70/1
  14DOF整车模型/32(Fx_rr) -> Goto71/1
  14DOF整车模型/33(Fy_rr) -> Goto72/1
  14DOF整车模型/34(Fz_rr) -> Goto73/1
  From69/1 -> Mux2/23
  From70/1 -> Mux2/24
  From71/1 -> Mux2/25
  From72/1 -> Mux2/26
  From73/1 -> Mux2/27
  From74/1 -> Mux2/28
  From75/1 -> Mux2/29
  From76/1 -> Mux2/30
  From77/1 -> Mux2/31
  From78/1 -> Mux2/32
  From79/1 -> Mux2/33
  From80/1 -> Mux2/34
  From81/1 -> To Workspace1/1
  From82/1 -> To Workspace3/1
  From83/1 -> To Workspace4/1
  From84/1 -> To Workspace5/1
  7DOF整车模型/17(Fy_rl) -> Goto84/1
  7DOF整车模型/10(Fx_fl) -> Goto77/1
  7DOF整车模型/19(Fx_rr) -> Goto86/1
  7DOF整车模型/21(Fz_rr) -> Goto88/1
  7DOF整车模型/14(Fy_fr) -> Goto81/1
  7DOF整车模型/11(Fy_fl) -> Goto78/1
  7DOF整车模型/12(Fz_fl) -> Goto79/1
  7DOF整车模型/20(Fy_rr) -> Goto87/1
  7DOF整车模型/13(Fx_fr) -> Goto80/1
  7DOF整车模型/18(Fz_rl) -> Goto85/1
  7DOF整车模型/16(Fx_rl) -> Goto83/1
  7DOF整车模型/15(Fz_fr) -> Goto82/1
  From88/1 -> Demux2/1
  Demux2/1 -> 7DOF整车模型/5(T_fl)
  Demux2/2 -> 7DOF整车模型/6(T_fr)
  Demux2/3 -> 7DOF整车模型/7(T_rl)
  Demux2/4 -> 7DOF整车模型/8(T_rr)
  Demux4/1 -> 7DOF整车模型/1(delta_fl)
  Demux4/2 -> 7DOF整车模型/2(delta_fr)
  Demux4/3 -> 7DOF整车模型/3(delta_rr)
  Demux4/4 -> 7DOF整车模型/4(delta_rl)
  From89/1 -> Demux4/1
  7DOF整车模型/9(beta_z) -> Goto90/1
  7DOF整车模型/8(ay) -> Goto89/1
  7DOF整车模型/1(x) -> Goto91/1
  7DOF整车模型/2(y) -> Goto92/1
  7DOF整车模型/3(yaw) -> Goto93/1
  7DOF整车模型/4(vx) -> Goto76/1
  7DOF整车模型/5(vy) -> Goto75/1
  7DOF整车模型/6(wz) -> Goto34/1
  7DOF整车模型/7(ax) -> Goto74/1
  From90/1 -> Mux3/1
  From91/1 -> Mux3/2
  Mux3/1 -> Goto94/1
  From87/1 -> To Workspace6/1
  7DOF整车模型/22(w_fl) -> Goto95/1
  7DOF整车模型/23(w_fr) -> Goto96/1
  7DOF整车模型/24(w_rl) -> Goto97/1
  7DOF整车模型/25(w_rr) -> Goto98/1
  From28/1 -> Mux3/10
  From29/1 -> Mux3/11
  From30/1 -> Mux3/12
  From85/1 -> Mux3/13
  From99/1 -> Mux3/14
  From100/1 -> Mux3/15
  From101/1 -> Mux3/16
  From102/1 -> Mux3/17
  From103/1 -> Mux3/18
  From104/1 -> Mux3/19
  From105/1 -> Mux3/20
  From106/1 -> Mux3/21
  From107/1 -> Mux3/22
  From108/1 -> Mux3/23
  From109/1 -> Mux3/24
  From110/1 -> Mux3/25
  Mux5/1 -> Goto99/1
  From113/1 -> Mux5/1
  From114/1 -> Mux5/2
  From116/1 -> Mux5/3
  From118/1 -> Mux5/4
  From119/1 -> Mux5/5
  From120/1 -> Mux5/6
  From124/1 -> Mux5/7
  From127/1 -> Mux5/8
  From130/1 -> Mux5/9
  From131/1 -> Mux5/10
  From132/1 -> Mux5/11
  From133/1 -> Mux5/12
  From134/1 -> Mux5/13
  From111/1 -> Mux5/14
  From112/1 -> Mux5/15
  From135/1 -> Mux5/16
  From136/1 -> Mux5/17
  From137/1 -> Mux5/18
  From138/1 -> Mux5/19
  From139/1 -> Mux5/20
  From140/1 -> Mux5/21
  From141/1 -> Mux5/22
  From142/1 -> Mux5/23
  From143/1 -> Mux5/24
  From144/1 -> Mux5/25
  From98/1 -> Mux3/9
  From95/1 -> Mux3/8
  From92/1 -> Mux3/7
  From97/1 -> Mux3/6
  From96/1 -> Mux3/5
  From94/1 -> Mux3/4
  From93/1 -> Mux3/3
  From117/1 -> Add1/1
  From115/1 -> Add1/2
  Add1/1 -> Goto100/1
  From123/1 -> To Workspace8/1
  From121/1 -> To Workspace2/1
  From122/1 -> To Workspace7/1
  3DOF整车模型/17(w_rl) -> Goto124/1
  Demux5/1 -> 3DOF整车模型/5(T_fl)
  3DOF整车模型/9(beta_z) -> Goto118/1
  3DOF整车模型/4(vx) -> Goto104/1
  Demux5/2 -> 3DOF整车模型/6(T_fr)
  From32/1 -> Demux6/1
  3DOF整车模型/6(wz) -> Goto101/1
  Demux6/3 -> 3DOF整车模型/3(delta_rr)
  3DOF整车模型/8(ay) -> Goto117/1
  Demux6/1 -> 3DOF整车模型/1(delta_fl)
  3DOF整车模型/16(w_fl) -> Goto122/1
  3DOF整车模型/3(yaw) -> Goto121/1
  3DOF整车模型/5(vy) -> Goto103/1
  Demux5/3 -> 3DOF整车模型/7(T_rl)
  3DOF整车模型/7(ax) -> Goto102/1
  From31/1 -> Demux5/1
  3DOF整车模型/1(x) -> Goto119/1
  Demux6/4 -> 3DOF整车模型/4(delta_rl)
  Demux6/2 -> 3DOF整车模型/2(delta_fr)
  Demux5/4 -> 3DOF整车模型/8(T_rr)
  3DOF整车模型/2(y) -> Goto120/1
  3DOF整车模型/10(Fx_fl) -> Gain11/1
  Gain11/1 -> Goto105/1
  3DOF整车模型/11(Fy_fl) -> Gain18/1
  Gain18/1 -> Goto106/1
  3DOF整车模型/12(Fz_fl) -> Gain19/1
  Gain19/1 -> Goto107/1
  3DOF整车模型/13(Fx_rl) -> Gain20/1
  Gain20/1 -> Goto111/1
  3DOF整车模型/14(Fy_rl) -> Gain21/1
  Gain21/1 -> Goto112/1
  3DOF整车模型/15(Fz_rl) -> Gain22/1
  Gain22/1 -> Goto113/1
  From161/1 -> Mux6/9
  From156/1 -> Mux6/3
  From157/1 -> Mux6/4
  From160/1 -> Mux6/6
  From155/1 -> Mux6/7
  From159/1 -> Mux6/5
  From158/1 -> Mux6/8
  From154/1 -> Mux6/2
  Mux6/1 -> Goto108/1
  From153/1 -> Mux6/1
  From149/1 -> Mux6/10, Mux6/11
  From151/1 -> Mux6/12, Mux6/13
  From162/1 -> Gain23/1
  Gain23/1 -> Mux6/14
  From33/1 -> Gain24/1
  Gain24/1 -> Mux6/15
  Gain25/1 -> Mux6/16
  From34/1 -> Gain25/1
  From86/1 -> Gain26/1
  From126/1 -> Gain28/1
  From125/1 -> Gain27/1
  Gain26/1 -> Mux6/17
  Gain27/1 -> Mux6/18
  Gain28/1 -> Mux6/19
  From145/1 -> Gain29/1
  From148/1 -> Gain32/1
  From147/1 -> Gain31/1
  From129/1 -> Gain34/1
  From146/1 -> Gain30/1
  From128/1 -> Gain33/1
  Gain30/1 -> Mux6/21
  Gain29/1 -> Mux6/20
  Gain32/1 -> Mux6/23
  Gain33/1 -> Mux6/24
  Gain31/1 -> Mux6/22
  Gain34/1 -> Mux6/25
  From152/1 -> Add2/2
  From163/1 -> Add2/1
  Add2/1 -> Goto109/1
  From164/1 -> To Workspace10/1
  From150/1 -> To Workspace9/1
  From166/1 -> XY Graph/2
  From165/1 -> XY Graph/1
  From167/1 -> XY Graph/3
  From168/1 -> XY Graph/4
  From169/1 -> XY Graph/5
  From170/1 -> XY Graph/6
  [x_trucksim] -> XY Graph/7
  [y_trucksim] -> XY Graph/8
  From173/1 -> Add3/1
  From174/1 -> Add3/2
  Add3/1 -> Scope/1
  Constant/1 -> Mux/4, Mux/3
  Demux1/3 -> Trucksim_Input/3
  Demux1/4 -> Trucksim_Input/4
  Demux1/5 -> Trucksim_Input/5
  Demux1/6 -> Trucksim_Input/6
  Trucksim_Input/1 -> TruckSim S-Function/1
  [T_motor] -> Demux3/1
  Demux3/1 -> Trucksim_Input/7
  Demux3/2 -> Trucksim_Input/8
  Demux3/3 -> Trucksim_Input/9
  Demux3/4 -> Trucksim_Input/10
  Demux3/5 -> Trucksim_Input/11
  Demux3/6 -> Trucksim_Input/12
  Gain4/1 -> [ax_trucksim]
  Gain5/1 -> [ay_trucksim]
  Gain3/1 -> [w_ml_trucksim]
  Gain6/1 -> [w_mr_trucksim]
  Trucksim_Output/1 -> Gain4/1
  Trucksim_Output/2 -> Gain5/1
  Trucksim_Output/3 -> [beta_z_trucksim]
  Trucksim_Output/4 -> Scope6/1, Gain/1
  Trucksim_Output/5 -> Gain2/1
  Trucksim_Output/6 -> Gain12/1
  Trucksim_Output/7 -> [x_trucksim]
  Trucksim_Output/8 -> [y_trucksim]
  Trucksim_Output/9 -> Gain9/1
  Trucksim_Output/10 -> Gain13/1
  Trucksim_Output/11 -> Gain14/1
  Trucksim_Output/12 -> Gain3/1
  Trucksim_Output/13 -> Gain6/1
  Trucksim_Output/14 -> Gain15/1
  Trucksim_Output/15 -> Gain16/1
  Trucksim_Output/16 -> Scope2/1, [Fx_fl_trucksim]
  Trucksim_Output/17 -> [Fx_fr_trucksim]
  Trucksim_Output/18 -> [Fx_ml_trucksim]
  Trucksim_Output/19 -> [Fx_mr_trucksim]
  Trucksim_Output/20 -> [Fx_rl_trucksim]
  Trucksim_Output/21 -> [Fx_rr_trucksim]
  Trucksim_Output/22 -> [Fy_fl_trucksim]
  Trucksim_Output/23 -> [Fy_fr_trucksim]
  Trucksim_Output/24 -> [Fy_ml_trucksim]
  Trucksim_Output/25 -> [Fy_mr_trucksim]
  Trucksim_Output/26 -> [Fy_rl_trucksim]
  Trucksim_Output/27 -> [Fy_rr_trucksim]
  Trucksim_Output/28 -> [Fz_fl_trucksim]
  Trucksim_Output/29 -> [Fz_fr_trucksim]
  Trucksim_Output/30 -> [Fz_ml_trucksim]
  Trucksim_Output/31 -> [Fz_mr_trucksim]
  Trucksim_Output/32 -> [Fz_rl_trucksim]
  Trucksim_Output/33 -> [Fz_rr_trucksim]
  [x_trucksim] -> Mux7/1
  [y_trucksim] -> Mux7/2
  [yaw_trucksim] -> Mux7/3
  [vx_trucksim] -> Mux7/4
  [vy_trucksim] -> Mux7/5
  [wz_trucksim] -> Mux7/6
  [ax_trucksim] -> Mux7/7
  [ay_trucksim] -> Mux7/8
  [beta_z_trucksim] -> Mux7/9
  [w_fl_trucksim] -> Mux7/10
  [w_fr_trucksim] -> Mux7/11
  [w_ml_trucksim] -> Mux7/12
  [w_mr_trucksim] -> Mux7/13
  [w_rl_trucksim] -> Mux7/14
  [w_rr_trucksim] -> Mux7/15
  [Fx_fl_trucksim] -> Mux7/16
  [Fx_fr_trucksim] -> Mux7/17
  [Fx_ml_trucksim] -> Mux7/18
  [Fx_mr_trucksim] -> Mux7/19
  [Fx_rl_trucksim] -> Mux7/20
  [Fx_rr_trucksim] -> Mux7/21
  [Fy_fl_trucksim] -> Mux7/22
  [Fy_fr_trucksim] -> Mux7/23
  [Fy_ml_trucksim] -> Mux7/24
  [Fy_mr_trucksim] -> Mux7/25
  [Fy_rl_trucksim] -> Mux7/26
  [Fy_rr_trucksim] -> Mux7/27
  [Fz_fl_trucksim] -> Mux7/28
  [Fz_fr_trucksim] -> Mux7/29
  [Fz_ml_trucksim] -> Mux7/30
  [Fz_mr_trucksim] -> Mux7/31
  [Fz_rl_trucksim] -> Mux7/32
  [Fz_rr_trucksim] -> Mux7/33
  Mux7/1 -> To Workspace11/1
  [T_motor] -> To Workspace12/1
  [delta_act] -> To Workspace13/1
  TruckSim S-Function/1 -> Trucksim_Output/1
  [Alpha_fl_trucksim] -> Mux7/34
  [Alpha_fr_trucksim] -> Mux7/35
  [Alpha_ml_trucksim] -> Mux7/36
  [Alpha_mr_trucksim] -> Mux7/37
  [Alpha_rl_trucksim] -> Mux7/38
  [Alpha_rr_trucksim] -> Mux7/39
  Trucksim_Output/34 -> Gain8/1
  Gain8/1 -> [Alpha_fl_trucksim]
  Trucksim_Output/35 -> Gain10/1
  Gain10/1 -> [Alpha_fr_trucksim]
  Trucksim_Output/36 -> Gain35/1
  Gain35/1 -> [Alpha_ml_trucksim]
  Trucksim_Output/37 -> Gain36/1
  Gain36/1 -> [Alpha_mr_trucksim]
  Trucksim_Output/38 -> Gain37/1
  Gain37/1 -> [Alpha_rl_trucksim]
  Trucksim_Output/39 -> Gain38/1
  Gain38/1 -> [Alpha_rr_trucksim]
  Gain39/1 -> Mux4/3
  Gain7/1 -> Mux4/2, Mux4/4, Mux4/6, Mux4/5, Gain39/1, Mux4/1, Scope5/1
  Mux9/1 -> [T_motor]
  Constant1/1 -> Mux8/4, Mux8/3
  Gain40/1 -> Mux8/6, Mux8/5
  Mux8/1 -> [delta_act]
  Gain42/1 -> Scope3/1, Mux9/1, Mux9/2, Mux9/3, Mux9/4, Mux9/6, Mux9/5
  Signal Editor-tank_turn/1 -> Mux/1, Gain1/1
  Gain43/1 -> Mux/6
  Signal Editor-tank_turn/2 -> Mux/2, Gain43/1
  Signal Editor-tank_turn/3 -> Gain7/1
  Signal Editor-opposite_steering/2 -> Gain40/1, Mux8/2, Scope1/1, Mux8/1
  Mux11/1 -> Goto128/1
  Constant3/1 -> Mux10/6, Mux10/5
  Gain44/1 -> Scope7/1, Mux11/2, Mux11/3, Mux11/4, Mux11/6, Mux11/5, Mux11/1
  Signal Editor-front_middle_steering/1 -> Gain44/1
  Signal Editor-front_middle_steering/2 -> Gain45/1, Mux10/2, Mux10/1, Scope4/1
  Mux10/1 -> Goto127/1
  Trigonometric Function1/1 -> Mux10/3, Mux10/4
  Mux12/1 -> Goto129/1
  Gain41/1 -> Scope9/1, Mux13/1, Mux13/2, Mux13/3, Mux13/4, Mux13/6, Mux13/5
  Mux13/1 -> Goto130/1
  Gain45/1 -> Trigonometric Function/1
  Trigonometric Function/1 -> Trigonometric Function1/1
  Constant2/1 -> Gain46/1, Mux12/6, Mux12/4, Mux12/2, Scope8/1
  Gain46/1 -> Mux12/5, Mux12/1, Mux12/3
  Signal Editor-same_steering_crab_motion/1 -> Gain41/1
  Signal Editor-lateral_movement/1 -> Gain47/1
  Mux15/1 -> Goto132/1
  Gain47/1 -> Gain50/1, Gain49/1, Scope11/1, Mux15/1, Mux15/3, Gain51/1, Mux15/5
  Mux14/1 -> Goto131/1
  Gain51/1 -> Mux15/6
  Gain50/1 -> Mux15/4
  Gain49/1 -> Mux15/2
  Constant4/1 -> Mux14/1, Mux14/3, Mux14/5, Gain53/1, Gain48/1, Gain52/1, Scope10/1
  Gain52/1 -> Mux14/2
  Gain53/1 -> Mux14/6
  Gain48/1 -> Mux14/4
  Signal Editor-lateral_movement/2 -> Terminator1/1
  Gain54/1 -> Scope13/1, Mux17/2, Mux17/3, Mux17/4, Mux17/6, Mux17/5, Mux17/1
  Signal Editor-only_front_steering/2 -> Mux16/2, Mux16/1, Scope12/1
  Mux17/1 -> Goto134/1
  Constant5/1 -> Mux16/6, Mux16/5
  Constant6/1 -> Mux16/3, Mux16/4
  Signal Editor-only_front_steering/1 -> Gain54/1
  Mux16/1 -> Goto133/1
  Signal Editor-opposite_steering/1 -> Gain42/1

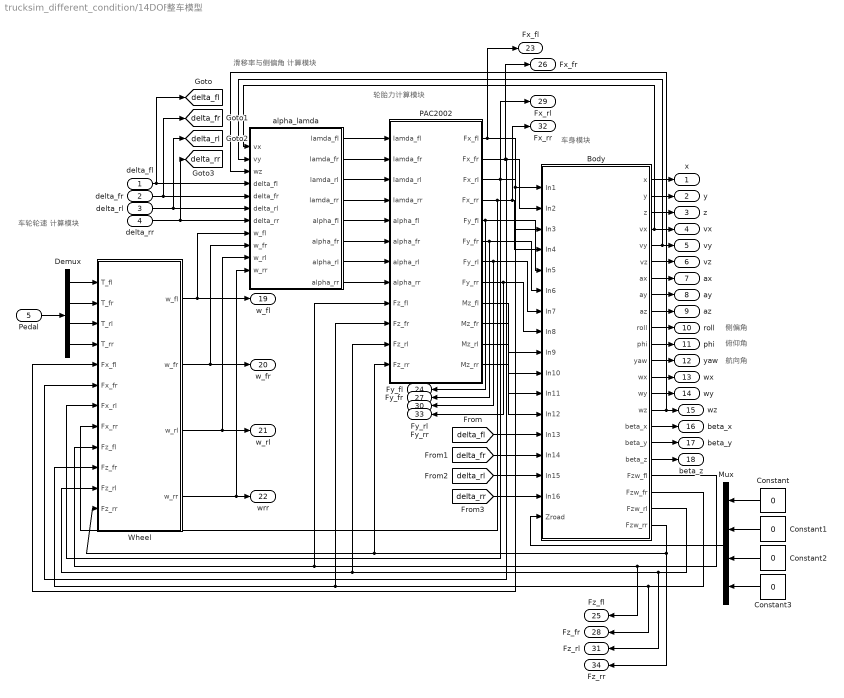
== system trucksim_different_condition/14DOF整车模型 ==
  note: 车身模块
  note: 航向角
  note: 侧偏角
  note: 俯仰角
  note: 轮胎力计算模块
  note: 滑移率与侧偏角
      | 计算模块
  note: 车轮轮速
      | 计算模块
  delta_fl : Inport
  delta_fr : Inport  Port=2
  delta_rl : Inport  Port=3
  delta_rr : Inport  Port=4
  Pedal : Inport  Port=5
  Body : Subsystem
  Constant{,1..3} (4 alike) : Constant  Value=0
  Demux : Demux
  Mux : Mux
  PAC2002 : Subsystem
  Wheel : Subsystem
  alpha_lamda : Subsystem
  x : Outport
  y : Outport  Port=2
  z : Outport  Port=3
  vx : Outport  Port=4
  vy : Outport  Port=5
  vz : Outport  Port=6
  ax : Outport  Port=7
  ay : Outport  Port=8
  az : Outport  Port=9
  roll : Outport  Port=10
  phi : Outport  Port=11
  yaw : Outport  Port=12
  wx : Outport  Port=13
  wy : Outport  Port=14
  wz : Outport  Port=15
  beta_x : Outport  Port=16
  beta_y : Outport  Port=17
  beta_z : Outport  Port=18
  w_fl : Outport  Port=19
  w_fr : Outport  Port=20
  w_rl : Outport  Port=21
  wrr : Outport  Port=22
  Fx_fl : Outport  Port=23
  Fy_fl : Outport  Port=24
  Fz_fl : Outport  Port=25
  Fx_fr : Outport  Port=26
  Fy_fr : Outport  Port=27
  Fz_fr : Outport  Port=28
  Fx_rl : Outport  Port=29
  Fy_rl : Outport  Port=30
  Fz_rl : Outport  Port=31
  Fx_rr : Outport  Port=32
  Fy_rr : Outport  Port=33
  Fz_rr : Outport  Port=34
  tag scope: delta_fl=global, delta_fr=global, delta_rl=global, delta_rr=global
  wires:
  delta_fl/1 -> alpha_lamda/4(delta_fl), [delta_fl]
  delta_rr/1 -> alpha_lamda/7(delta_rr), [delta_rr]
  delta_fr/1 -> alpha_lamda/5(delta_fr), [delta_fr]
  delta_rl/1 -> [delta_rl], alpha_lamda/6(delta_rl)
  alpha_lamda/1(lamda_fl) -> PAC2002/1(lamda_fl)
  alpha_lamda/7(alpha_rl) -> PAC2002/7(alpha_rl)
  Wheel/2(w_fr) -> w_fr/1, alpha_lamda/9(w_fr)
  PAC2002/5(Fy_fl) -> Body/5(In5), Fy_fl/1
  alpha_lamda/2(lamda_fr) -> PAC2002/2(lamda_fr)
  alpha_lamda/5(alpha_fl) -> PAC2002/5(alpha_fl)
  alpha_lamda/3(lamda_rl) -> PAC2002/3(lamda_rl)
  alpha_lamda/4(lamda_rr) -> PAC2002/4(lamda_rr)
  PAC2002/9(Mz_fl) -> Body/9(In9)
  PAC2002/10(Mz_fr) -> Body/10(In10)
  Wheel/4(w_rr) -> alpha_lamda/11(w_rr), wrr/1
  PAC2002/4(Fx_rr) -> Fx_rr/1, Body/4(In4), Wheel/8(Fx_rr)
  alpha_lamda/6(alpha_fr) -> PAC2002/6(alpha_fr)
  PAC2002/3(Fx_rl) -> Fx_rl/1, Body/3(In3), Wheel/7(Fx_rl)
  Wheel/3(w_rl) -> w_rl/1, alpha_lamda/10(w_rl)
  PAC2002/7(Fy_rl) -> Fy_rl/1, Body/7(In7)
  PAC2002/2(Fx_fr) -> Body/2(In2), Wheel/6(Fx_fr), Fx_fr/1
  PAC2002/8(Fy_rr) -> Fy_rr/1, Body/8(In8)
  alpha_lamda/8(alpha_rr) -> PAC2002/8(alpha_rr)
  PAC2002/1(Fx_fl) -> Wheel/5(Fx_fl), Body/1(In1), Fx_fl/1
  PAC2002/12(Mz_rr) -> Body/12(In12)
  Demux/3 -> Wheel/3(T_rl)
  Demux/2 -> Wheel/2(T_fr)
  Demux/1 -> Wheel/1(T_fl)
  PAC2002/11(Mz_rl) -> Body/11(In11)
  Demux/4 -> Wheel/4(T_rr)
  PAC2002/6(Fy_fr) -> Fy_fr/1, Body/6(In6)
  Pedal/1 -> Demux/1
  [delta_fl] -> Body/13(In13)
  [delta_fr] -> Body/14(In14)
  [delta_rl] -> Body/15(In15)
  [delta_rr] -> Body/16(In16)
  Mux/1 -> Body/17(Zroad)
  Body/1(x) -> x/1
  Body/2(y) -> y/1
  Body/3(z) -> z/1
  Body/4(vx) -> vx/1, alpha_lamda/1(vx)
  Body/5(vy) -> alpha_lamda/2(vy), vy/1
  Body/6(vz) -> vz/1
  Body/7(ax) -> ax/1
  Body/8(ay) -> ay/1
  Body/9(az) -> az/1
  Body/10(roll) -> roll/1
  Body/11(phi) -> phi/1
  Body/12(yaw) -> yaw/1
  Body/13(wx) -> wx/1
  Body/16(beta_x) -> beta_x/1
  Body/14(wy) -> wy/1
  Body/15(wz) -> alpha_lamda/3(wz), wz/1
  Body/18(beta_z) -> beta_z/1
  Body/19(Fzw_fl) -> Fz_fl/1, PAC2002/9(Fz_fl), Wheel/9(Fz_fl)
  Body/20(Fzw_fr) -> Fz_fr/1, PAC2002/10(Fz_fr), Wheel/10(Fz_fr)
  Body/21(Fzw_rl) -> Fz_rl/1, Wheel/11(Fz_rl), PAC2002/11(Fz_rl)
  Body/22(Fzw_rr) -> Fz_rr/1, PAC2002/12(Fz_rr), Wheel/12(Fz_rr)
  Wheel/1(w_fl) -> w_fl/1, alpha_lamda/8(w_fl)
  Body/17(beta_y) -> beta_y/1
  Constant/1 -> Mux/1
  Constant1/1 -> Mux/2
  Constant2/1 -> Mux/3
  Constant3/1 -> Mux/4

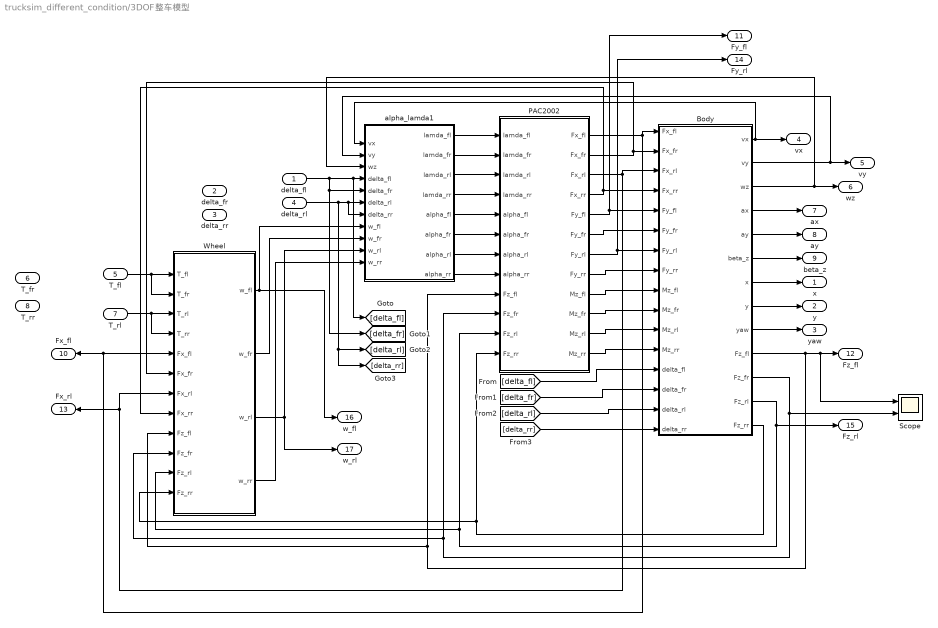
== system trucksim_different_condition/3DOF整车模型 ==
  delta_fl : Inport
  delta_fr : Inport  Port=2
  delta_rr : Inport  Port=3
  delta_rl : Inport  Port=4
  T_fl : Inport  Port=5
  T_fr : Inport  Port=6
  T_rl : Inport  Port=7
  T_rr : Inport  Port=8
  Body : Subsystem
  PAC2002 : Subsystem
  Scope : Scope  NumInputPorts=2
  Wheel : Subsystem
  alpha_lamda1 : Subsystem
  x : Outport
  y : Outport  Port=2
  yaw : Outport  Port=3
  vx : Outport  Port=4
  vy : Outport  Port=5
  wz : Outport  Port=6
  ax : Outport  Port=7
  ay : Outport  Port=8
  beta_z : Outport  Port=9
  Fx_fl : Outport  Port=10
  Fy_fl : Outport  Port=11
  Fz_fl : Outport  Port=12
  Fx_rl : Outport  Port=13
  Fy_rl : Outport  Port=14
  Fz_rl : Outport  Port=15
  w_fl : Outport  Port=16
  w_rl : Outport  Port=17
  wires:
  PAC2002/12(Mz_rr) -> Body/12(Mz_rr)
  PAC2002/11(Mz_rl) -> Body/11(Mz_rl)
  PAC2002/10(Mz_fr) -> Body/10(Mz_fr)
  PAC2002/9(Mz_fl) -> Body/9(Mz_fl)
  T_rl/1 -> Wheel/4(T_rr), Wheel/3(T_rl)
  Body/1(vx) -> vx/1, alpha_lamda1/1(vx)
  Body/2(vy) -> vy/1, alpha_lamda1/2(vy)
  T_fl/1 -> Wheel/1(T_fl), Wheel/2(T_fr)
  Body/13(Fz_rr) -> PAC2002/12(Fz_rr), Wheel/12(Fz_rr)
  PAC2002/3(Fx_rl) -> Fx_rl/1, Wheel/7(Fx_rl), Body/3(Fx_rl)
  alpha_lamda1/6(alpha_fr) -> PAC2002/6(alpha_fr)
  Body/11(Fz_fr) -> Scope/2, PAC2002/10(Fz_fr), Wheel/10(Fz_fr)
  [delta_fr] -> Body/14(delta_fr)
  alpha_lamda1/5(alpha_fl) -> PAC2002/5(alpha_fl)
  alpha_lamda1/8(alpha_rr) -> PAC2002/8(alpha_rr)
  Wheel/3(w_rl) -> w_rl/1, alpha_lamda1/10(w_rl)
  Body/12(Fz_rl) -> Fz_rl/1, PAC2002/11(Fz_rl), Wheel/11(Fz_rl)
  alpha_lamda1/7(alpha_rl) -> PAC2002/7(alpha_rl)
  PAC2002/8(Fy_rr) -> Body/8(Fy_rr)
  alpha_lamda1/2(lamda_fr) -> PAC2002/2(lamda_fr)
  PAC2002/5(Fy_fl) -> Fy_fl/1, Body/5(Fy_fl)
  PAC2002/2(Fx_fr) -> Wheel/6(Fx_fr), Body/2(Fx_fr)
  Body/10(Fz_fl) -> Scope/1, Fz_fl/1, PAC2002/9(Fz_fl), Wheel/9(Fz_fl)
  alpha_lamda1/3(lamda_rl) -> PAC2002/3(lamda_rl)
  PAC2002/6(Fy_fr) -> Body/6(Fy_fr)
  PAC2002/7(Fy_rl) -> Fy_rl/1, Body/7(Fy_rl)
  alpha_lamda1/4(lamda_rr) -> PAC2002/4(lamda_rr)
  alpha_lamda1/1(lamda_fl) -> PAC2002/1(lamda_fl)
  PAC2002/1(Fx_fl) -> Fx_fl/1, Wheel/5(Fx_fl), Body/1(Fx_fl)
  [delta_fl] -> Body/13(delta_fl)
  Body/3(wz) -> wz/1, alpha_lamda1/3(wz)
  PAC2002/4(Fx_rr) -> Wheel/8(Fx_rr), Body/4(Fx_rr)
  Body/4(ax) -> ax/1
  Wheel/2(w_fr) -> alpha_lamda1/9(w_fr)
  Wheel/1(w_fl) -> w_fl/1, alpha_lamda1/8(w_fl)
  Wheel/4(w_rr) -> alpha_lamda1/11(w_rr)
  delta_fl/1 -> [delta_fl], alpha_lamda1/4(delta_fl), [delta_fr], alpha_lamda1/5(delta_fr)
  delta_rl/1 -> [delta_rl], [delta_rr], alpha_lamda1/7(delta_rr), alpha_lamda1/6(delta_rl)
  Body/7(x) -> x/1
  Body/8(y) -> y/1
  Body/5(ay) -> ay/1
  Body/9(yaw) -> yaw/1
  Body/6(beta_z) -> beta_z/1
  [delta_rl] -> Body/15(delta_rl)
  [delta_rr] -> Body/16(delta_rr)

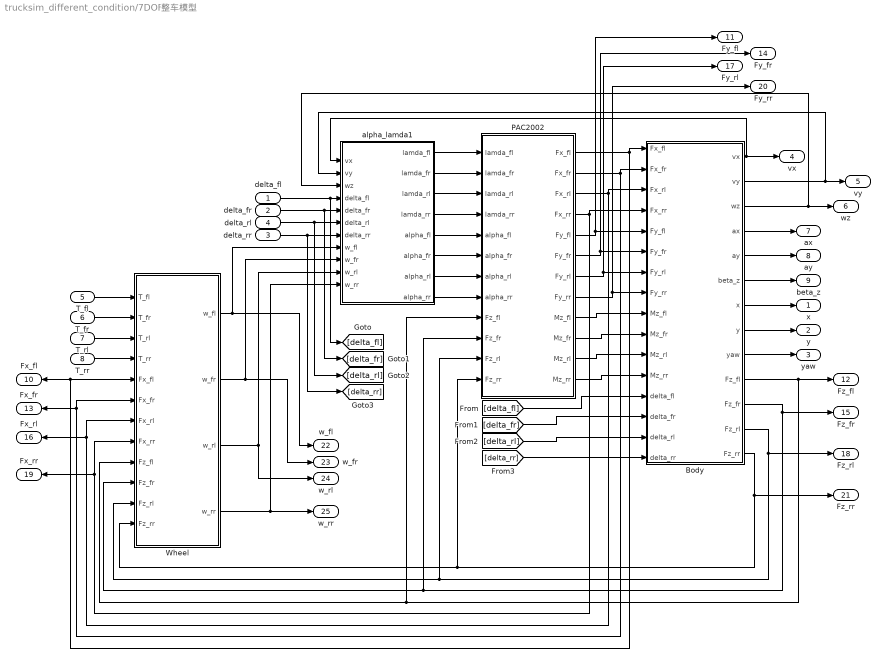
== system trucksim_different_condition/7DOF整车模型 ==
  delta_fl : Inport
  delta_fr : Inport  Port=2
  delta_rr : Inport  Port=3
  delta_rl : Inport  Port=4
  T_fl : Inport  Port=5
  T_fr : Inport  Port=6
  T_rl : Inport  Port=7
  T_rr : Inport  Port=8
  Body : Subsystem
  PAC2002 : Subsystem
  Wheel : Subsystem
  alpha_lamda1 : Subsystem
  x : Outport
  y : Outport  Port=2
  yaw : Outport  Port=3
  vx : Outport  Port=4
  vy : Outport  Port=5
  wz : Outport  Port=6
  ax : Outport  Port=7
  ay : Outport  Port=8
  beta_z : Outport  Port=9
  Fx_fl : Outport  Port=10
  Fy_fl : Outport  Port=11
  Fz_fl : Outport  Port=12
  Fx_fr : Outport  Port=13
  Fy_fr : Outport  Port=14
  Fz_fr : Outport  Port=15
  Fx_rl : Outport  Port=16
  Fy_rl : Outport  Port=17
  Fz_rl : Outport  Port=18
  Fx_rr : Outport  Port=19
  Fy_rr : Outport  Port=20
  Fz_rr : Outport  Port=21
  w_fl : Outport  Port=22
  w_fr : Outport  Port=23
  w_rl : Outport  Port=24
  w_rr : Outport  Port=25
  wires:
  PAC2002/12(Mz_rr) -> Body/12(Mz_rr)
  PAC2002/11(Mz_rl) -> Body/11(Mz_rl)
  PAC2002/10(Mz_fr) -> Body/10(Mz_fr)
  PAC2002/9(Mz_fl) -> Body/9(Mz_fl)
  T_rr/1 -> Wheel/4(T_rr)
  T_rl/1 -> Wheel/3(T_rl)
  Body/1(vx) -> vx/1, alpha_lamda1/1(vx)
  Body/2(vy) -> vy/1, alpha_lamda1/2(vy)
  T_fl/1 -> Wheel/1(T_fl)
  Body/13(Fz_rr) -> PAC2002/12(Fz_rr), Wheel/12(Fz_rr), Fz_rr/1
  T_fr/1 -> Wheel/2(T_fr)
  PAC2002/3(Fx_rl) -> Fx_rl/1, Wheel/7(Fx_rl), Body/3(Fx_rl)
  alpha_lamda1/6(alpha_fr) -> PAC2002/6(alpha_fr)
  Body/11(Fz_fr) -> Fz_fr/1, PAC2002/10(Fz_fr), Wheel/10(Fz_fr)
  [delta_fr] -> Body/14(delta_fr)
  alpha_lamda1/5(alpha_fl) -> PAC2002/5(alpha_fl)
  alpha_lamda1/8(alpha_rr) -> PAC2002/8(alpha_rr)
  Wheel/3(w_rl) -> w_rl/1, alpha_lamda1/10(w_rl)
  Body/12(Fz_rl) -> Fz_rl/1, PAC2002/11(Fz_rl), Wheel/11(Fz_rl)
  alpha_lamda1/7(alpha_rl) -> PAC2002/7(alpha_rl)
  PAC2002/8(Fy_rr) -> Fy_rr/1, Body/8(Fy_rr)
  alpha_lamda1/2(lamda_fr) -> PAC2002/2(lamda_fr)
  PAC2002/5(Fy_fl) -> Fy_fl/1, Body/5(Fy_fl)
  PAC2002/2(Fx_fr) -> Fx_fr/1, Wheel/6(Fx_fr), Body/2(Fx_fr)
  Body/10(Fz_fl) -> Fz_fl/1, PAC2002/9(Fz_fl), Wheel/9(Fz_fl)
  alpha_lamda1/3(lamda_rl) -> PAC2002/3(lamda_rl)
  PAC2002/6(Fy_fr) -> Fy_fr/1, Body/6(Fy_fr)
  PAC2002/7(Fy_rl) -> Fy_rl/1, Body/7(Fy_rl)
  alpha_lamda1/4(lamda_rr) -> PAC2002/4(lamda_rr)
  alpha_lamda1/1(lamda_fl) -> PAC2002/1(lamda_fl)
  PAC2002/1(Fx_fl) -> Fx_fl/1, Wheel/5(Fx_fl), Body/1(Fx_fl)
  [delta_fl] -> Body/13(delta_fl)
  Body/3(wz) -> wz/1, alpha_lamda1/3(wz)
  PAC2002/4(Fx_rr) -> Fx_rr/1, Wheel/8(Fx_rr), Body/4(Fx_rr)
  Body/4(ax) -> ax/1
  Wheel/2(w_fr) -> w_fr/1, alpha_lamda1/9(w_fr)
  Wheel/1(w_fl) -> w_fl/1, alpha_lamda1/8(w_fl)
  Wheel/4(w_rr) -> w_rr/1, alpha_lamda1/11(w_rr)
  delta_fl/1 -> [delta_fl], alpha_lamda1/4(delta_fl)
  delta_fr/1 -> alpha_lamda1/5(delta_fr), [delta_fr]
  delta_rl/1 -> [delta_rl], alpha_lamda1/6(delta_rl)
  delta_rr/1 -> alpha_lamda1/7(delta_rr), [delta_rr]
  Body/7(x) -> x/1
  Body/8(y) -> y/1
  Body/5(ay) -> ay/1
  Body/9(yaw) -> yaw/1
  Body/6(beta_z) -> beta_z/1
  [delta_rl] -> Body/15(delta_rl)
  [delta_rr] -> Body/16(delta_rr)
